simulink model "ModelGroup15"  (R2026b)
settings: Solver=VariableStepAuto  StopTime=inf
settings Model: Creator=khols  LastModifiedBy=khols

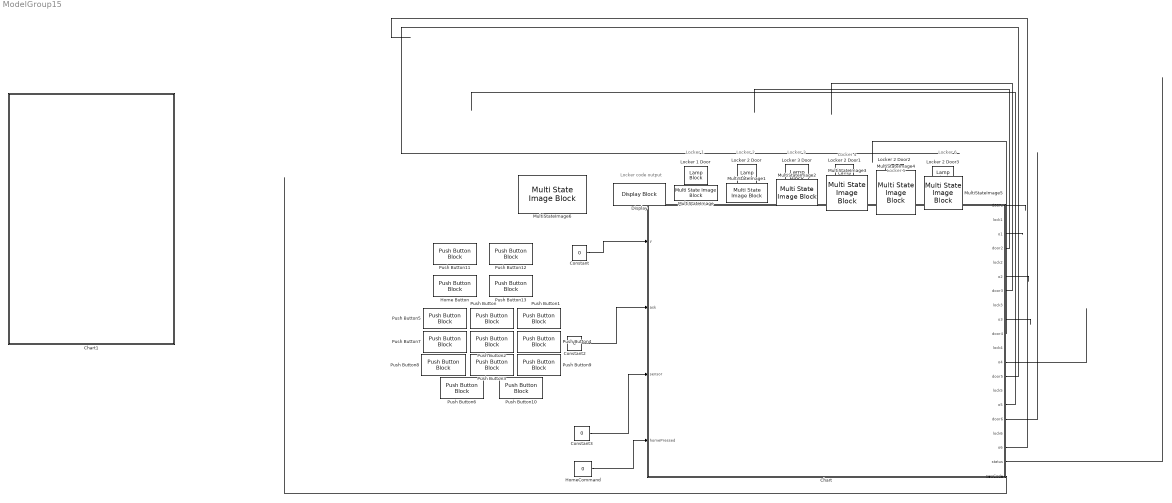
== system ModelGroup15 ==
  note: Locker 4
  note: Locker 2
  note: Locker 5
  note: Locker 6
  note: Locker 3
  note: Locker 1
  note: Locker code output
  Chart : Stateflow chart  TreatAsAtomicUnit=on
      settings: PortSchema="{\"entries\":[{\"content\":{\"sides\":[{\"content\":{\"connectorIds\":[\"In1\",\"In2\",\"In3\",\"In4\"]},\"type\":\"ConnectorPlacement.EquallySpacedRectSide\",\"uuid\":\"1e3907da-80ef-450c-96ba-243d945a5803\"},{\"content\":{\"connectorIds\":[\"Out1\",\"Out2\",\"Out13\",\"Out3\",\"Out4\",\"Out14\",\"Out5\",\"Out6\",\"Out15\",\"Out7\",\"Out8\",\"Out16\",\"Out9\",\"Out10\",\"Out17\",\"Out11\",\"Out12\",\"Out18\",\"Out19\",\"Out20\"],\"side\":\"RIGHT\"},\"type\":\"ConnectorPlacement.EquallySpacedRectSide\",\"uuid\":\"121ad9a2-3887-491d-8c30-9fd70d9375d7\"},{\"content\":{\"side\":\"TOP\"},\"type\":\"ConnectorPlacement.EquallySpacedRectSide\",\"uuid\":\"11a18cae-b11d-4403-b37b-259055059525\"}]},\"type\":\"ConnectorPlacement.EquallySpacedConnector\",\"uuid\":\"3a7c1146-386a-4ebb-ae09-1c69c9d75140\"}],\"packageUris\":[\"http://schema.mathworks.com/mf0/Connector/R2020b\"],\"version\":\"1.0\"}"
  Chart1 : Stateflow chart  TreatAsAtomicUnit=on
  Constant : Constant  Value=0  VectorParams1D=off  SampleTime=0.05
  Constant2 : Constant  Value=0
  Constant3 : Constant  Value=0
  Display : DisplayBlock  LabelPosition=Hide  Transparency=1  GridColor=[0.502, 0.502, 0.502]
  Home Button : PushButtonBlock  ButtonText=Home  IconOnColor=[0.0, 0.39215686274509803, 0.0]  IconOffColor=[0.0, 1.0, 0.0]  OffValue=0.000000
  HomeCommand : Constant  Value=0
  Locker 1 Door : LampBlock  LabelPosition=Hide  DefaultColor=[192.0, 192.0, 192.0]
  Locker 2 Door{,1..3} (4 alike) : LampBlock  LabelPosition=Hide  DefaultColor=[192.0, 192.0, 192.0]
  Locker 3 Door : LampBlock  LabelPosition=Hide  DefaultColor=[192.0, 192.0, 192.0]
  MultiStateImage{,1..6} (7 alike) : MultiStateImageBlock  LabelPosition=Hide
  Push Button : PushButtonBlock  ButtonText=2  OnValue=2  IconOnColor=[0.0, 0.39215686274509803, 0.0]  IconOffColor=[0.0, 1.0, 0.0]  OffValue=0.000000
  Push Button1 : PushButtonBlock  ButtonText=3  OnValue=3  IconOnColor=[0.0, 0.39215686274509803, 0.0]  IconOffColor=[0.0, 1.0, 0.0]  OffValue=0.000000
  Push Button10 : PushButtonBlock  ButtonText=*  OnValue=11  IconOnColor=[0.0, 0.39215686274509803, 0.0]  IconOffColor=[0.0, 1.0, 0.0]  OffValue=0.000000
  Push Button11 : PushButtonBlock  ButtonText=Store  IconOnColor=[0.0, 0.39215686274509803, 0.0]  IconOffColor=[0.0, 1.0, 0.0]  OffValue=0.000000
  Push Button12 : PushButtonBlock  ButtonText=Retreive  OnValue=2  IconOnColor=[0.0, 0.39215686274509803, 0.0]  IconOffColor=[0.0, 1.0, 0.0]  OffValue=0.000000
  Push Button13 : PushButtonBlock  ButtonText=Input Item  IconOnColor=[0.0, 0.39215686274509803, 0.0]  IconOffColor=[0.0, 1.0, 0.0]  OffValue=0.000000
  Push Button2 : PushButtonBlock  ButtonText=5  OnValue=5  IconOnColor=[0.0, 0.39215686274509803, 0.0]  IconOffColor=[0.0, 1.0, 0.0]  OffValue=0.000000
  Push Button3 : PushButtonBlock  ButtonText=8  OnValue=8  IconOnColor=[0.0, 0.39215686274509803, 0.0]  IconOffColor=[0.0, 1.0, 0.0]  OffValue=0.000000
  Push Button4 : PushButtonBlock  ButtonText=6  OnValue=6  IconOnColor=[0.0, 0.39215686274509803, 0.0]  IconOffColor=[0.0, 1.0, 0.0]  OffValue=0.000000
  Push Button5 : PushButtonBlock  ButtonText=1  IconOnColor=[0.0, 0.39215686274509803, 0.0]  IconOffColor=[0.0, 1.0, 0.0]  OffValue=0.000000
  Push Button6 : PushButtonBlock  ButtonText=#  OnValue=10  IconOnColor=[0.0, 0.39215686274509803, 0.0]  IconOffColor=[0.0, 1.0, 0.0]  OffValue=0.000000
  Push Button7 : PushButtonBlock  ButtonText=4  OnValue=4  IconOnColor=[0.0, 0.39215686274509803, 0.0]  IconOffColor=[0.0, 1.0, 0.0]  OffValue=0.000000
  Push Button8 : PushButtonBlock  ButtonText=7  OnValue=7  IconOnColor=[0.0, 0.39215686274509803, 0.0]  IconOffColor=[0.0, 1.0, 0.0]  OffValue=0.000000
  Push Button9 : PushButtonBlock  ButtonText=9  OnValue=9  IconOnColor=[0.0, 0.39215686274509803, 0.0]  IconOffColor=[0.0, 1.0, 0.0]  OffValue=0.000000
  wires:
  Constant/1 -> Chart/1(y)
  Constant2/1 -> Chart/2(ask)
  Constant3/1 -> Chart/3(sensor)
  Chart/1(door1) -> ?
  Chart/3(door2) -> ?
  Chart/5(door3) -> ?
  Chart/7(door4) -> ?
  Chart/9(door5) -> ?
  Chart/11(door6) -> ?
  Chart/13(o1) -> ?
  Chart/14(o2) -> ?
  Chart/15(o3) -> ?
  Chart/16(o4) -> ?
  Chart/17(o5) -> ?
  Chart/18(o6) -> ?
  Chart/19(status) -> ?
  HomeCommand/1 -> Chart/4(homePressed)
  Chart/20(newCode) -> ?

== stateflow chart ModelGroup15/Chart1 ==

== stateflow chart ModelGroup15/Chart ==
  state enteredCodeLogic [parallel]
    settings: executionOrder=1
    state awaitCode
    state awaitDigit1
    state awaitDigit7
    state awaitDigit8
    state awaitDigit2
    state reset
      d1=0
      d2=0
      d3=0
      d4=0
    state awaitDigit3
    state awaitDigit6
    state awaitDigit4
    state awaitDigit5
    state compileCode3
      entry:
      if (isequal(maintainanceCode,[d1 d2 d3 d4]))
      if maintain == 0
      maintain = 1;
      else
      maintain = 0;
      end
      end
    state compileCode2
      enteredCode = [d1 d2 d3 d4];
    (default) -> awaitCode
    awaitCode -> awaitDigit1 [order 1] : [y==11]
    awaitCode -> awaitDigit7 [order 2] : [y==10&&retrieval == 1]
    awaitDigit1 -> reset [order 2] : [homePressed == 1 || after(15,sec)]
    awaitDigit7 -> reset [order 2] : [homePressed == 1 || after(15,sec)]
    awaitDigit1 -> awaitDigit2 [order 1] : [hasChangedFrom(y,0) && y >= 1 && y <= 9]{d1=y}
    reset -> awaitCode : after(1,tick)
    awaitDigit7 -> awaitDigit8 [order 1] : [hasChangedFrom(y,0) && y >= 1 && y <= 9]{d1=y}
    awaitDigit8 -> reset [order 2] : [homePressed == 1 || after(15,sec)]
    awaitDigit2 -> reset [order 2] : [homePressed == 1 || after(15,sec)]
    awaitDigit3 -> reset [order 2] : [homePressed == 1 || after(15,sec)]
    awaitDigit6 -> reset [order 2] : [homePressed == 1 || after(15,sec)]
    awaitDigit8 -> awaitDigit6 [order 1] : [hasChangedFrom(y,0) && y >= 1 && y <= 9]{d2=y}
    awaitDigit2 -> awaitDigit3 [order 1] : [hasChangedFrom(y,0) && y >= 1 && y <= 9]{d2=y}
    awaitDigit5 -> reset [order 2] : [homePressed == 1 || after(15,sec)]
    awaitDigit4 -> reset [order 2] : [homePressed == 1 || after(15,sec)]
    awaitDigit3 -> awaitDigit4 [order 1] : [hasChangedFrom(y,0) && y >= 1 && y <= 9]{d3=y}
    awaitDigit6 -> awaitDigit5 [order 1] : [hasChangedFrom(y,0) && y >= 1 && y <= 9]{d3=y}
    awaitDigit4 -> compileCode3 [order 1] : [hasChangedFrom(y,0) && y >= 1 && y <= 9]{d4=y}
    awaitDigit5 -> compileCode2 [order 1] : [hasChangedFrom(y,0) && y >= 1 && y <= 9]{d4=y}
    compileCode2 -> enteredCodeLogic : after(1,sec)
    compileCode3 -> enteredCodeLogic : after(1,sec)
  state Main [parallel]
    settings: executionOrder=2
    state ParcelLogic
      state entry
        entry:
        retrieval = 0
        status = 0;
      state AwaitReset
      state ParcelRetrieval1
        entry:
        parcelDetected = 1;
        state WaitForRemoval
        state OpenDoor
          entry:
          door1 = 1;
        state UnlockDoor
          entry:
          lock1 = 0;
        state CloseDoor
          entry:
          door1= 0;
        state LockDoor
          entry:
          lock1 =1;
          status = 4;
        (default) -> Main.ParcelLogic.ParcelRetrieval1.UnlockDoor
        Main.ParcelLogic.ParcelRetrieval1.UnlockDoor -> Main.ParcelLogic.ParcelRetrieval1.OpenDoor
        Main.ParcelLogic.ParcelRetrieval1.OpenDoor -> Main.ParcelLogic.ParcelRetrieval1.WaitForRemoval : after(1,sec)
        Main.ParcelLogic.ParcelRetrieval1.WaitForRemoval -> Main.ParcelLogic.ParcelRetrieval1.CloseDoor [order 2] : [sensor==0]{parcelDetected=0;}
        Main.ParcelLogic.ParcelRetrieval1.WaitForRemoval -> Main.ParcelLogic.ParcelRetrieval1.CloseDoor [order 1] : after(15,sec)
        Main.ParcelLogic.ParcelRetrieval1.CloseDoor -> Main.ParcelLogic.ParcelRetrieval1.LockDoor : after(1,sec)
      state StorageFull
        entry:
        status = 6;
      state ParcelStorage1
        entry:
        parcelDetected = 0;
        en, du:
        state WaitForParcel
        state UnlockDoor
          en:
          lock1 = 0;
        state OpenDoor
          entry:
          door1 = 1;
        state GenerateCode1
          entry:
          newCode = generateCode(1);
          while isequal(newCode,code1) || isequal(newCode,code2) || ...
          isequal(newCode,code3) || isequal(newCode,code4) || ...
          isequal(newCode,code5) || isequal(newCode,code6)
          newCode = generateCode(1);
          end
          code1 = newCode;
          o1 = 1;
        state LockDoor
          entry:
          lock1 =1;
          status = 2;
        state CloseDoor
          entry:
          door1 = 0;
        (default) -> Main.ParcelLogic.ParcelStorage1.UnlockDoor
        Main.ParcelLogic.ParcelStorage1.OpenDoor -> Main.ParcelLogic.ParcelStorage1.WaitForParcel
        Main.ParcelLogic.ParcelStorage1.WaitForParcel -> Main.ParcelLogic.ParcelStorage1.CloseDoor [order 1] : after(15,sec)
        Main.ParcelLogic.ParcelStorage1.WaitForParcel -> Main.ParcelLogic.ParcelStorage1.CloseDoor [order 2] : [sensor==1]{parcelDetected=1;}
        Main.ParcelLogic.ParcelStorage1.UnlockDoor -> Main.ParcelLogic.ParcelStorage1.OpenDoor
        Main.ParcelLogic.ParcelStorage1.CloseDoor -> Main.ParcelLogic.ParcelStorage1.LockDoor
        Main.ParcelLogic.ParcelStorage1.LockDoor -> GenerateCode1 [order 1] : [parcelDetected==1 && after(1,sec)]
      state Store
        during:
        l=o1 && o2 && o3 && o4 && o5 && o6;
        status = 1;
      state Retrieval
        if ~isequal(enteredCode,baseCode)&&operationComplete==false
        if isequal(enteredCode,code1)
        activeDoor=1
        failedCode=0
        end
        if isequal(enteredCode,code2)
        activeDoor=2
        failedCode=0
        end
        if isequal(enteredCode,code3)
        activeDoor=3
        failedCode=0
        end
        if isequal(enteredCode,code4)
        activeDoor=4
        failedCode=0
        end
        if isequal(enteredCode,code5)
        activeDoor=5
        failedCode=0
        end
        if isequal(enteredCode,code6)
        activeDoor=6
        failedCode=0
        end
        end
        status = 3;
      state ParcelRetrieval2
        entry:
        parcelDetected = 1;
        state WaitForRemoval
        state OpenDoor
          entry:
          door2 = 1;
        state UnlockDoor
          entry:
          lock2 = 0;
        state CloseDoor
          entry:
          door2= 0;
        state LockDoor
          entry:
          lock2 =1;
          status = 4;
        (default) -> Main.ParcelLogic.ParcelRetrieval2.UnlockDoor
        Main.ParcelLogic.ParcelRetrieval2.UnlockDoor -> Main.ParcelLogic.ParcelRetrieval2.OpenDoor
        Main.ParcelLogic.ParcelRetrieval2.OpenDoor -> Main.ParcelLogic.ParcelRetrieval2.WaitForRemoval : after(1,sec)
        Main.ParcelLogic.ParcelRetrieval2.WaitForRemoval -> Main.ParcelLogic.ParcelRetrieval2.CloseDoor [order 2] : [sensor==0]{parcelDetected=0;}
        Main.ParcelLogic.ParcelRetrieval2.WaitForRemoval -> Main.ParcelLogic.ParcelRetrieval2.CloseDoor [order 1] : after(15,sec)
        Main.ParcelLogic.ParcelRetrieval2.CloseDoor -> Main.ParcelLogic.ParcelRetrieval2.LockDoor : after(1,sec)
      state ParcelStorage2
        entry:
        parcelDetected=0;
        en, du:
        state UnlockDoor
          en:
          lock2 = 0;
        state OpenDoor
          entry:
          door2 = 1;
        state WaitForParcel
        state GenerateCode2
          entry:
          newCode = generateCode(2);
          while isequal(newCode,code1) || isequal(newCode,code2) || ...
          isequal(newCode,code3) || isequal(newCode,code4) || ...
          isequal(newCode,code5) || isequal(newCode,code6)
          newCode = generateCode(2);
          end
          code2 = newCode;
          o2 = 1;
        state LockDoor
          entry:
          lock2 =1;
          status = 2;
        state CloseDoor
          entry:
          door2 = 0;
        (default) -> Main.ParcelLogic.ParcelStorage2.UnlockDoor
        Main.ParcelLogic.ParcelStorage2.UnlockDoor -> Main.ParcelLogic.ParcelStorage2.OpenDoor
        Main.ParcelLogic.ParcelStorage2.OpenDoor -> Main.ParcelLogic.ParcelStorage2.WaitForParcel
        Main.ParcelLogic.ParcelStorage2.WaitForParcel -> Main.ParcelLogic.ParcelStorage2.CloseDoor [order 1] : after(15,sec)
        Main.ParcelLogic.ParcelStorage2.WaitForParcel -> Main.ParcelLogic.ParcelStorage2.CloseDoor [order 2] : [sensor==1]{parcelDetected=1;}
        Main.ParcelLogic.ParcelStorage2.LockDoor -> GenerateCode2 [order 2] : [parcelDetected==1 && after(1,sec)]
        Main.ParcelLogic.ParcelStorage2.CloseDoor -> Main.ParcelLogic.ParcelStorage2.LockDoor
      state ParcelRetrieval3
        entry:
        parcelDetected = 1;
        state WaitForRemoval
        state OpenDoor
          entry:
          door3 = 1;
        state UnlockDoor
          entry:
          lock3 = 0;
        state CloseDoor
          entry:
          door3= 0;
        state LockDoor
          entry:
          lock3 =1;
          status = 4;
        (default) -> Main.ParcelLogic.ParcelRetrieval3.UnlockDoor
        Main.ParcelLogic.ParcelRetrieval3.UnlockDoor -> Main.ParcelLogic.ParcelRetrieval3.OpenDoor
        Main.ParcelLogic.ParcelRetrieval3.OpenDoor -> Main.ParcelLogic.ParcelRetrieval3.WaitForRemoval : after(1,sec)
        Main.ParcelLogic.ParcelRetrieval3.WaitForRemoval -> Main.ParcelLogic.ParcelRetrieval3.CloseDoor [order 2] : [sensor==0]{parcelDetected=0;}
        Main.ParcelLogic.ParcelRetrieval3.WaitForRemoval -> Main.ParcelLogic.ParcelRetrieval3.CloseDoor [order 1] : after(15,sec)
        Main.ParcelLogic.ParcelRetrieval3.CloseDoor -> Main.ParcelLogic.ParcelRetrieval3.LockDoor : after(1,sec)
      state ParcelStorage3
        entry:
        parcelDetected=0;
        en, du:
        state OpenDoor
          entry:
          door3 = 1;
        state WaitForParcel
        state UnlockDoor
          en:
          lock3 = 0;
        state GenerateCode3
          entry:
          newCode = generateCode(3);
          while isequal(newCode,code1) || isequal(newCode,code2) || ...
          isequal(newCode,code3) || isequal(newCode,code4) || ...
          isequal(newCode,code5) || isequal(newCode,code6)
          newCode = generateCode(3);
          end
          code3 = newCode;
          o3 = 1;
        state CloseDoor
          entry:
          door3 = 0;
        state LockDoor
          entry:
          lock3 =1;
          status = 2;
        (default) -> Main.ParcelLogic.ParcelStorage3.UnlockDoor
        Main.ParcelLogic.ParcelStorage3.UnlockDoor -> Main.ParcelLogic.ParcelStorage3.OpenDoor
        Main.ParcelLogic.ParcelStorage3.OpenDoor -> Main.ParcelLogic.ParcelStorage3.WaitForParcel
        Main.ParcelLogic.ParcelStorage3.WaitForParcel -> Main.ParcelLogic.ParcelStorage3.CloseDoor [order 1] : after(15,sec)
        Main.ParcelLogic.ParcelStorage3.WaitForParcel -> Main.ParcelLogic.ParcelStorage3.CloseDoor [order 2] : [sensor==1]{parcelDetected=1;}
        Main.ParcelLogic.ParcelStorage3.CloseDoor -> Main.ParcelLogic.ParcelStorage3.LockDoor
        Main.ParcelLogic.ParcelStorage3.LockDoor -> GenerateCode3 [order 2] : [parcelDetected==1 && after(1,sec)]
      state ParcelRetrieval4
        entry:
        parcelDetected = 1;
        state WaitForRemoval
        state OpenDoor
          entry:
          door4 = 1;
        state UnlockDoor
          entry:
          lock4 = 0;
        state CloseDoor
          entry:
          door4= 0;
        state LockDoor
          entry:
          lock4 =1;
          status = 4;
        (default) -> Main.ParcelLogic.ParcelRetrieval4.UnlockDoor
        Main.ParcelLogic.ParcelRetrieval4.UnlockDoor -> Main.ParcelLogic.ParcelRetrieval4.OpenDoor
        Main.ParcelLogic.ParcelRetrieval4.OpenDoor -> Main.ParcelLogic.ParcelRetrieval4.WaitForRemoval : after(1,sec)
        Main.ParcelLogic.ParcelRetrieval4.WaitForRemoval -> Main.ParcelLogic.ParcelRetrieval4.CloseDoor [order 2] : [sensor==0]{parcelDetected=0;}
        Main.ParcelLogic.ParcelRetrieval4.WaitForRemoval -> Main.ParcelLogic.ParcelRetrieval4.CloseDoor [order 1] : after(15,sec)
        Main.ParcelLogic.ParcelRetrieval4.CloseDoor -> Main.ParcelLogic.ParcelRetrieval4.LockDoor : after(1,sec)
      state ParcelStorage4
        entry:
        parcelDetected=0;
        en, du:
        state OpenDoor
          entry:
          door4 = 1;
        state WaitForParcel
        state UnlockDoor
          en:
          lock4 = 0;
        state GenerateCode4
          entry:
          newCode = generateCode(4);
          while isequal(newCode,code1) || isequal(newCode,code2) || ...
          isequal(newCode,code3) || isequal(newCode,code4) || ...
          isequal(newCode,code5) || isequal(newCode,code6)
          newCode = generateCode(4);
          end
          code4 = newCode;
          o4 = 1;
        state LockDoor
          entry:
          lock4 =1;
          status = 2;
        state CloseDoor
          entry:
          door4 = 0;
        (default) -> Main.ParcelLogic.ParcelStorage4.UnlockDoor
        Main.ParcelLogic.ParcelStorage4.UnlockDoor -> Main.ParcelLogic.ParcelStorage4.OpenDoor
        Main.ParcelLogic.ParcelStorage4.OpenDoor -> Main.ParcelLogic.ParcelStorage4.WaitForParcel
        Main.ParcelLogic.ParcelStorage4.WaitForParcel -> Main.ParcelLogic.ParcelStorage4.CloseDoor [order 2] : [sensor==1]{parcelDetected=1;}
        Main.ParcelLogic.ParcelStorage4.WaitForParcel -> Main.ParcelLogic.ParcelStorage4.CloseDoor [order 1] : after(15,sec)
        Main.ParcelLogic.ParcelStorage4.CloseDoor -> Main.ParcelLogic.ParcelStorage4.LockDoor
        Main.ParcelLogic.ParcelStorage4.LockDoor -> GenerateCode4 [order 2] : [parcelDetected==1 && after(1,sec)]
      state ParcelRetrieval5
        entry:
        parcelDetected = 1;
        state WaitForRemoval
        state OpenDoor
          entry:
          door5 = 1;
        state UnlockDoor
          entry:
          lock5 = 0;
        state CloseDoor
          entry:
          door5= 0;
        state LockDoor
          entry:
          lock5 =1;
          status = 4;
        (default) -> Main.ParcelLogic.ParcelRetrieval5.UnlockDoor
        Main.ParcelLogic.ParcelRetrieval5.UnlockDoor -> Main.ParcelLogic.ParcelRetrieval5.OpenDoor
        Main.ParcelLogic.ParcelRetrieval5.OpenDoor -> Main.ParcelLogic.ParcelRetrieval5.WaitForRemoval : after(1,sec)
        Main.ParcelLogic.ParcelRetrieval5.WaitForRemoval -> Main.ParcelLogic.ParcelRetrieval5.CloseDoor [order 2] : [sensor==0]{parcelDetected=0;}
        Main.ParcelLogic.ParcelRetrieval5.WaitForRemoval -> Main.ParcelLogic.ParcelRetrieval5.CloseDoor [order 1] : after(15,sec)
        Main.ParcelLogic.ParcelRetrieval5.CloseDoor -> Main.ParcelLogic.ParcelRetrieval5.LockDoor : after(1,sec)
      state ParcelStorage5
        entry:
        parcelDetected=0;
        en, du:
        state UnlockDoor
          en:
          lock5 = 0;
        state OpenDoor
          entry:
          door5 = 1;
        state WaitForParcel
        state GenerateCode5
          entry:
          newCode = generateCode(5);
          while isequal(newCode,code1) || isequal(newCode,code2) || ...
          isequal(newCode,code3) || isequal(newCode,code4) || ...
          isequal(newCode,code5) || isequal(newCode,code6)
          newCode = generateCode(5);
          end
          code5 = newCode;
          o5 = 1;
        state LockDoor
          entry:
          lock5 =1;
          status = 2;
        state CloseDoor
          entry:
          door5 = 0;
        (default) -> Main.ParcelLogic.ParcelStorage5.UnlockDoor
        Main.ParcelLogic.ParcelStorage5.OpenDoor -> Main.ParcelLogic.ParcelStorage5.WaitForParcel
        Main.ParcelLogic.ParcelStorage5.UnlockDoor -> Main.ParcelLogic.ParcelStorage5.OpenDoor
        Main.ParcelLogic.ParcelStorage5.WaitForParcel -> Main.ParcelLogic.ParcelStorage5.CloseDoor [order 1] : after(15,sec)
        Main.ParcelLogic.ParcelStorage5.WaitForParcel -> Main.ParcelLogic.ParcelStorage5.CloseDoor [order 2] : [sensor==1]{parcelDetected=1;}
        Main.ParcelLogic.ParcelStorage5.LockDoor -> GenerateCode5 [order 2] : [parcelDetected==1 && after(1,sec)]
        Main.ParcelLogic.ParcelStorage5.CloseDoor -> Main.ParcelLogic.ParcelStorage5.LockDoor
      state ParcelRetrieval6
        entry:
        parcelDetected = 1;
        state WaitForRemoval
        state OpenDoor
          entry:
          door6 = 1;
        state UnlockDoor
          entry:
          lock6 = 0;
        state CloseDoor
          entry:
          door6= 0;
        state LockDoor
          entry:
          lock6 =1;
          status = 4;
        (default) -> Main.ParcelLogic.ParcelRetrieval6.UnlockDoor
        Main.ParcelLogic.ParcelRetrieval6.UnlockDoor -> Main.ParcelLogic.ParcelRetrieval6.OpenDoor
        Main.ParcelLogic.ParcelRetrieval6.OpenDoor -> Main.ParcelLogic.ParcelRetrieval6.WaitForRemoval : after(1,sec)
        Main.ParcelLogic.ParcelRetrieval6.WaitForRemoval -> Main.ParcelLogic.ParcelRetrieval6.CloseDoor [order 2] : [sensor==0]{parcelDetected=0;}
        Main.ParcelLogic.ParcelRetrieval6.WaitForRemoval -> Main.ParcelLogic.ParcelRetrieval6.CloseDoor [order 1] : after(15,sec)
        Main.ParcelLogic.ParcelRetrieval6.CloseDoor -> Main.ParcelLogic.ParcelRetrieval6.LockDoor : after(1,sec)
      state ParcelStorage6
        entry:
        parcelDetected=0;
        en, du:
        state UnlockDoor
          en:
          lock6 = 0;
        state OpenDoor
          entry:
          door6 = 1;
        state WaitForParcel
        state GenerateCode6
          entry:
          newCode = generateCode(6);
          while isequal(newCode,code1) || isequal(newCode,code2) || ...
          isequal(newCode,code3) || isequal(newCode,code4) || ...
          isequal(newCode,code5) || isequal(newCode,code6)
          newCode = generateCode(6);
          end
          code6 = newCode;
          o6 = 1;
        state LockDoor
          entry:
          lock6 =1;
          status = 2;
        state CloseDoor
          entry:
          door6 = 0;
        (default) -> Main.ParcelLogic.ParcelStorage6.UnlockDoor
        Main.ParcelLogic.ParcelStorage6.OpenDoor -> Main.ParcelLogic.ParcelStorage6.WaitForParcel
        Main.ParcelLogic.ParcelStorage6.UnlockDoor -> Main.ParcelLogic.ParcelStorage6.OpenDoor
        Main.ParcelLogic.ParcelStorage6.WaitForParcel -> Main.ParcelLogic.ParcelStorage6.CloseDoor [order 1] : after(15,sec)
        Main.ParcelLogic.ParcelStorage6.WaitForParcel -> Main.ParcelLogic.ParcelStorage6.CloseDoor [order 2] : [sensor==1]{parcelDetected=1;}
        Main.ParcelLogic.ParcelStorage6.LockDoor -> GenerateCode6 [order 2] : [parcelDetected==1 && after(1,sec)]
        Main.ParcelLogic.ParcelStorage6.CloseDoor -> Main.ParcelLogic.ParcelStorage6.LockDoor
      state FailCheck
      (default) -> entry : {enteredCode=baseCode}
      Retrieval -> entry [order 9] : [homePressed == 1 && activeDoor == 0]{enteredCode = baseCode; operationComplete = false;}
      entry -> Retrieval [order 2] : [ask==2 && activeDoor==0]{retrieval=1}
      AwaitReset -> entry : [ask==0]{operationComplete=false; enteredCode=baseCode;}
      Store -> entry [order 8] : [homePressed == 1 && activeDoor == 0]{enteredCode = baseCode; operationComplete = false;}
      entry -> Store [order 1] : [ask==1 && activeDoor==0]
      StorageFull -> AwaitReset : after(2,sec)
      Retrieval -> AwaitReset [order 7] : [operationComplete==true && activeDoor==0]
      Store -> AwaitReset [order 9] : [operationComplete==true && activeDoor==0]
      Store -> StorageFull [order 1] : [ l==1]
      Retrieval -> ParcelRetrieval1 [order 6] : [o1==1 && operationComplete==false && activeDoor == 1]
      Store -> ParcelStorage1 [order 2] : [y==1&&o1==0&& activeDoor==0 && operationComplete==false]{activeDoor=1;}
      Main.ParcelLogic.ParcelRetrieval1.LockDoor -> Retrieval [order 1] : [parcelDetected==0 && after(1,sec)]/{o1=0; code1=baseCode; l=false; activeDoor=0;operationComplete = true;}
      GenerateCode1 -> Store : {activeDoor=0;operationComplete = true;}
      Main.ParcelLogic.ParcelRetrieval1.LockDoor -> Retrieval [order 2] : [parcelDetected==1 && after(1,sec)]/{o1=1; activeDoor=0;operationComplete = true;}
      Main.ParcelLogic.ParcelStorage1.LockDoor -> Store [order 2] : [parcelDetected==0 && after(1,sec)]/{o1=0; activeDoor=0;operationComplete = true;}
      Store -> ParcelStorage2 [order 6] : [y==2&&o2==0&& activeDoor==0 && operationComplete==false]{activeDoor=2;}
      Retrieval -> ParcelRetrieval2 [order 5] : [o2==1 && operationComplete==false && activeDoor == 2]
      Main.ParcelLogic.ParcelRetrieval2.LockDoor -> Retrieval [order 1] : [parcelDetected==1 && after(1,sec)]/{o2=1; activeDoor=0;operationComplete = true;}
      GenerateCode2 -> Store : {activeDoor=0;operationComplete = true;}
      Main.ParcelLogic.ParcelRetrieval2.LockDoor -> Retrieval [order 2] : [parcelDetected==0 && after(1,sec)]/{o2=0; code2=baseCode; l=false; activeDoor=0;operationComplete = true;}
      Main.ParcelLogic.ParcelStorage2.LockDoor -> Store [order 1] : [parcelDetected==0 && after(1,sec)]/{o2=0; l=o1&&o2&&o3&&o4&&o5&&o6; activeDoor=0;operationComplete = true;}
      Retrieval -> ParcelRetrieval3 [order 4] : [o3==1 && operationComplete==false && activeDoor == 3]
      Store -> ParcelStorage3 [order 7] : [y==3&&o3==0&& activeDoor==0 && operationComplete==false]{activeDoor=3;}
      GenerateCode3 -> Store : {l=o1&&o2&&o3&&o4&&o5&&o6; activeDoor=0;operationComplete = true;}
      Main.ParcelLogic.ParcelRetrieval3.LockDoor -> Retrieval [order 1] : [parcelDetected==1 && after(1,sec)]/{o3=1; activeDoor=0;operationComplete = true;}
      Main.ParcelLogic.ParcelRetrieval3.LockDoor -> Retrieval [order 2] : [parcelDetected==0 && after(1,sec)]/{o3=0; code3=baseCode; l=false; activeDoor=0;operationComplete = true;}
      Main.ParcelLogic.ParcelStorage3.LockDoor -> Store [order 1] : [parcelDetected==0 && after(1,sec)]/{o3=0; l=o1&&o2&&o3&&o4&&o5&&o6; activeDoor=0;operationComplete = true;}
      Store -> ParcelStorage4 [order 3] : [y==4&&o4==0&& activeDoor==0 && operationComplete==false]{activeDoor=4;}
      GenerateCode4 -> Store : {l=o1&&o2&&o3&&o4&&o5&&o6; activeDoor=0;operationComplete = true;}
      Retrieval -> ParcelRetrieval4 [order 3] : [o4==1 && operationComplete==false  && activeDoor == 4]
      Main.ParcelLogic.ParcelRetrieval4.LockDoor -> Retrieval [order 1] : [parcelDetected==0 && after(1,sec)]/{o4=0; code4=baseCode; l=false; activeDoor=0;operationComplete = true;}
      Main.ParcelLogic.ParcelStorage4.LockDoor -> Store [order 1] : [parcelDetected==0 && after(1,sec)]/{o4=0; l=o1&&o2&&o3&&o4&&o5&&o6; activeDoor=0;operationComplete = true;}
      Main.ParcelLogic.ParcelRetrieval4.LockDoor -> Retrieval [order 2] : [parcelDetected==1 && after(1,sec)]/{o4=1; activeDoor=0;operationComplete = true;}
      Store -> ParcelStorage5 [order 4] : [y==5&&o5==0&& activeDoor==0 && operationComplete==false]{activeDoor=5;}
      Retrieval -> ParcelRetrieval5 [order 2] : [o5==1 && operationComplete==false  && activeDoor == 5]
      GenerateCode5 -> Store : {l=o1&&o2&&o3&&o4&&o5&&o6; activeDoor=0;operationComplete = true;}
      Main.ParcelLogic.ParcelRetrieval5.LockDoor -> Retrieval [order 1] : [parcelDetected==0 && after(1,sec)]/{o5=0; code5=baseCode; l=false; activeDoor=0;operationComplete = true;}
      Main.ParcelLogic.ParcelStorage5.LockDoor -> Store [order 1] : [parcelDetected==0 && after(1,sec)]/{o5=0; l=o1&&o2&&o3&&o4&&o5&&o6; activeDoor=0;operationComplete = true;}
      Main.ParcelLogic.ParcelRetrieval5.LockDoor -> Retrieval [order 2] : [parcelDetected==1 && after(1,sec)]/{o5=1; activeDoor=0;operationComplete = true;}
      Retrieval -> ParcelRetrieval6 [order 1] : [o6==1 && operationComplete==false  && activeDoor == 6]
      Store -> ParcelStorage6 [order 5] : [y==6&&o6==0&& activeDoor==0 && operationComplete==false]{activeDoor=6;}
      Main.ParcelLogic.ParcelRetrieval6.LockDoor -> Retrieval [order 1] : [parcelDetected==0 && after(1,sec)]/{o6=0; code6=baseCode; l=false; activeDoor=0;operationComplete = true;}
      GenerateCode6 -> Store : {l=o1&&o2&&o3&&o4&&o5&&o6; activeDoor=0;operationComplete = true;}
      Main.ParcelLogic.ParcelRetrieval6.LockDoor -> Retrieval [order 2] : [parcelDetected==1 && after(1,sec)]/{o6=1; activeDoor=0;operationComplete = true;}
      Main.ParcelLogic.ParcelStorage6.LockDoor -> Store [order 1] : [parcelDetected==0 && after(1,sec)]/{o6=0; l=o1&&o2&&o3&&o4&&o5&&o6; activeDoor=0;operationComplete = true;}
      Retrieval -> FailCheck [order 8] : [~isequal(enteredCode, baseCode) && ...
          |  ~isequal(enteredCode, code1) && ...
          |  ~isequal(enteredCode, code2) && ...
          |  ~isequal(enteredCode, code3) && ...
          |  ~isequal(enteredCode, code4) && ...
          |  ~isequal(enteredCode, code5) && ...
          |  ~isequal(enteredCode, code6)]
      FailCheck -> Retrieval : after(1, sec){enteredCode=baseCode; failedCode = failedCode + 1;}
    state MaintainanceMode
      activeDoor=0;
      door1=0;
      door2=0;
      door3=0;
      door4=0;
      door5=0;
      door6=0;
      lock1=1;
      lock2=1;
      lock3=1;
      lock4=1;
      lock5=1;
      lock6=1;
    (default) -> ParcelLogic
    ParcelLogic -> MaintainanceMode [order 2] : [failedCode>=3]{maintain=2}
    ParcelLogic -> MaintainanceMode [order 1] : [maintain==1]
    MaintainanceMode -> ParcelLogic [order 1] : [maintain==0]{failedCode=0;}
    MaintainanceMode -> ParcelLogic [order 2] : after(15,sec)[maintain==2]{maintain=0; failedCode=0;}
  data: candidate function_output; nr function_input; enteredCode function_input; Hey function_output; y input; ask input; l local =false; sensor input; door1 output =0; lock1 output =1; door2 output =0; lock2 output =1; activeDoor local =0; door3 output =0; lock3 output =1; door4 output =0; lock4 output =1; door5 output =0; lock5 output =1; door6 output =0; lock6 output =1; parcelDetected local =0; code2 local =0 0 0 0; code3 local =0 0 0 0; code4 local =0 0 0 0; code5 local =0 0 0 0; code6 local =0 0 0 0; operationComplete local =false; failedCode local =0; maintain local =0; enteredCode local =0 0 0 0; maintainanceCode local =9 9 9 8; d1 local; d2 local; d3 local; d4 local; retrieval local =0; baseCode local =0 0 0 0; o1 output =0; o2 output =0; o3 output =0; o4 output =0; o5 output =0; o6 output =0; status output; homePressed input; code1 local = 0 0 0 0; newCode output =0 0 0 0
  function candidate = generateCode(nr):
    | function candidate = generateCode(nr)
    | coder.extrinsic('disp');
    | 
    | candidate = [randi([1, 9]), randi([1, 9]),randi([1, 9]),  randi([1, 9])];
    | 
    | fprintf('the code for box nr %d = [%d %d %d %d]\n', int32(nr), int32(candidate(1)), int32(candidate(2)), int32(candidate(3)), int32(candidate(4)))
    | end
  function Hey = checkCode(enteredCode):
    | function Hey = checkCode(enteredCode)
    | if (enteredCode == code1)
    |     lock1 = 0
    | end
